simulink model "Field_Control_DC_Shunt_Motor"  (R2023a)
settings: Solver=VariableStepAuto  StartTime=0.0  StopTime=10.0  RelTol=1e-3
libraries: spsDCMachineLib x1, spsDCVoltageSourceLib x1, spsSeriesRLCBranchLib x1, spspowerguiLib x1
settings Model: Creator=bolt  LastModifiedBy=monat
settings SolverCC: AlgebraicLoopSolver=TrustRegion
settings DebuggingCC: UnconnectedInputMsg=warning  UnconnectedOutputMsg=warning  UnconnectedLineMsg=warning
settings ModelReferenceCC: EnableRefExpFcnMdlSchedulingChecks=on

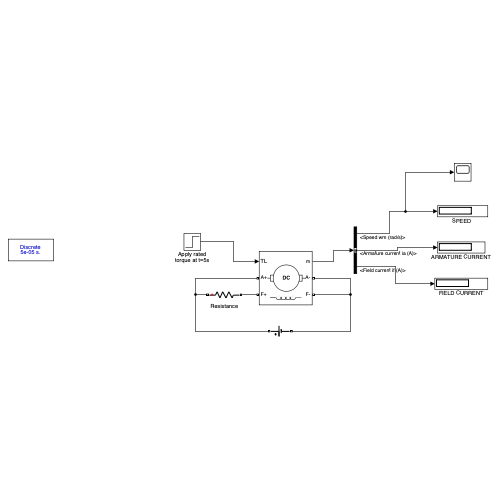
[thumbnail: Simulink's stored preview of the top-level diagram]
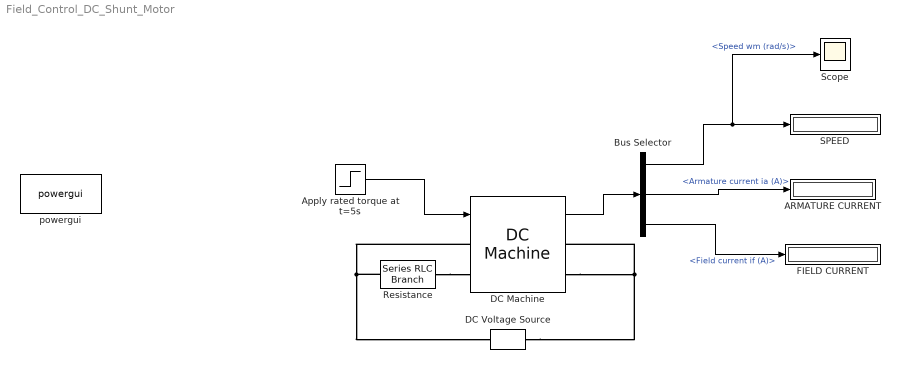
== system Field_Control_DC_Shunt_Motor ==
  ARMATURE CURRENT : Display
  Apply rated torque at t=5s : Step  Time=3  After=70%-0.25% -0.119  SampleTime=0
  Bus Selector : BusSelector  OutputSignals=Speed wm (rad/s),Armature current ia (A),Field current if (A)
  DC Machine : spsDCMachineLib/DC Machine  PresetModel=No  MechanicalLoad=Torque TL  FieldType=Wound  ShowDetailedParameters=on  MeasurementBus=off  RLa="[ 0.6  0.012]"  RLf="[ 240  120]"  Laf=1.8  MachineConstant=Torque constant (N.m/A)  Ke=1.8  Kt=1.8  J=1  Bm=0  Tf=0  w0=1  Ifinit=0.884615384615385  TsPowergui=0  TsBlock=-1
  DC Voltage Source : spsDCVoltageSourceLib/DC Voltage Source  Amplitude=230  Measurements=None
  FIELD CURRENT : Display
  Resistance : spsSeriesRLCBranchLib/Series RLC Branch  LConnTagsString=__new0  RConnTagsString=__new0  BranchType=R  Resistance=20  Inductance=1e-3  SetiL0=off  InitialCurrent=0  Capacitance=1e-6  Setx0=off  InitialVoltage=0  Measurements=None
  "SPEED " : Display
  Scope : Scope
  powergui : spspowerguiLib/powergui  Priority=1  SimulationMode=Discrete  SampleTime=50e-6  frequency=60  Iterations=50  frequencyindice=0  Pbase=100e6  ErrMax=1e-4  UnitsV=kV  UnitsW=MW  buscounter=0  FunctionMessages=off  echomessages=off  EnableUseOfTLC=off  CurrentSourceSwitches=off  DisableSnubberDevices=off  DisableRonSwitches=off  DisableVfSwitches=off  DisplayEquations=off  AutomaticDiscreteSolvers=off  SolverType=Tustin/Backward Euler (TBE)  Interpol=off  ExternalGateDelay=off  methode=off  Ts=100  x0status=blocks  SPID=on  SwTol=0  HookPort=off  NonlinearTolerance=1e-4  nMaxIteration=100  ContinueOnMaxIteration=off  RestoreLinks=warning  ResistiveCurrentMeasurement=off  Frange=[0:2:500]  Ylog=off  Xlog=on  ShowGrid=off  save=off  variable=ZData  structure=0  ZoomFFT=off  StartTime=0.0  cycles=1  DisplayStyle=1  fundamental=60  FreqAxis=off  MaxFrequency=1000  frequencyindicesteady=1  RmsSteady=1  display=off
  wires:
  Apply rated torque at t=5s/1 -> DC Machine/1
  DC Machine/1 -> Bus Selector/1
  Bus Selector/1 -> Scope/1, "SPEED "/1  "<Speed wm (rad/s)>"
  Bus Selector/2 -> ARMATURE CURRENT/1  "<Armature current ia (A)>"
  Bus Selector/3 -> FIELD CURRENT/1  "<Field current if (A)>"
  connections:
  Resistance/RConn1 -- DC Machine/LConn2
  Resistance/LConn1 -- DC Machine/LConn1 -- DC Voltage Source/RConn1
  DC Voltage Source/LConn1 -- DC Machine/RConn2 -- DC Machine/RConn1
